simulink model "sf_msg_traffic_light"  (R2025b)
settings: Solver=FixedStepDiscrete  StartTime=0.0  StopTime=inf  FixedStep=.2  RelTol=1e-3  EnableMultiTasking=on
PostLoadFcn:
  | tl_gui('init', bdroot);
InitFcn:
  | tl_gui('reset', bdroot);
libraries: sf_msg_traffic_light_lib x6
CloseFcn:
  | tl_gui('close');
settings Model: PacingRate=0.500000  Creator=The MathWorks, Inc.  LastModifiedBy=The MathWorks, Inc.
settings SolverCC: AlgebraicLoopSolver=TrustRegion
settings DataIOCC: LimitDataPoints=on  SaveOutput=off  SignalLogging=off  DSMLogging=off  SaveTime=off  ReturnWorkspaceOutputs=off
settings OptimizationCC: ReuseModelBlockBuffer=off  LifeSpan=inf
settings DebuggingCC: UnconnectedInputMsg=warning  UnconnectedOutputMsg=warning  UnconnectedLineMsg=warning  AllowSymbolicDim=off  PregeneratedLibrarySubsystemCodeDiagnostic=none  SFUnexpectedBacktrackingDiag=warning  SFNoUnconditionalDefaultTransitionDiag=warning  SFExecutionAtInitializationDiag=none  ArithmeticOperatorsInVariantConditions=warning
settings HardwareCC: ProdBitPerPointer=32.0  ProdBitPerSizeT=32.0  ProdBitPerPtrDiffT=32.0  ProdLargestAtomicFloat=None  ProdIntDivRoundTo=Undefined  ProdEndianess=Unspecified  ProdWordSize=32.0  ProdHWDeviceType=32-bit Generic
settings ModelReferenceCC: EnableRefExpFcnMdlSchedulingChecks=on  PropagateSignalLabelsOutOfModel=off
settings SFSimCC: SimUseLocalCustomCode=off  CustomCodeUndefinedFunction=UseInterfaceOnly
settings RTWCC: GenCodeOnly=on  GenerateReport=on  RTWUseLocalCustomCode=off  LaunchReport=on  GPUComputeCapability=3.5
settings CodeAppCC: StateflowObjectComments=on
settings GRTTargetCC: TargetLangStandard=C89/C90 (ANSI)  UtilityFuncGeneration=Shared location
settings ConfigComp: CovMetricSettings=dw  CovSaveCumulativeToWorkspaceVar=on  CovSaveSingleToWorkspaceVar=on  CovExternalEMLEnable=off

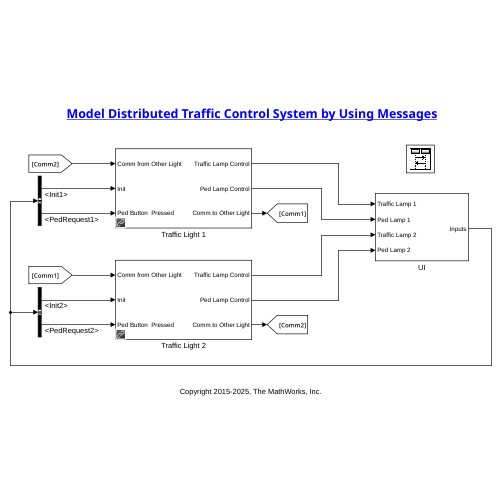
[thumbnail: Simulink's stored preview of the top-level diagram]
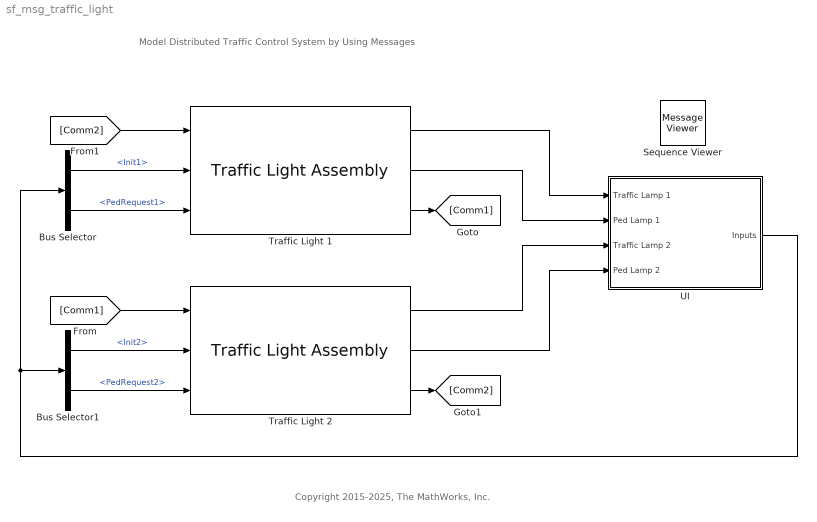
== system sf_msg_traffic_light ==
  note: Copyright 2015-2025, The MathWorks, Inc.
  note: Model Distributed Traffic Control System by Using Messages
  Bus Selector : BusSelector  OutputSignals=Init1,PedRequest1
  Bus Selector1 : BusSelector  OutputSignals=Init2,PedRequest2
  Sequence Viewer : MessageViewer  SavedRootId=#
  Traffic Light 1 : sf_msg_traffic_light_lib/Traffic Light Assembly  SystemSampleTime=-1  VariantActivationTime=update diagram  EmptyChoice=off  PassThrough=off  PassThroughVariantControl=(default)  EmptyChoiceVariantControl=(default)  AllowFlexibleInterface=on  Latency=0  AutoFrameSizeCalculation=off
  Traffic Light 2 : sf_msg_traffic_light_lib/Traffic Light Assembly  SystemSampleTime=-1  VariantActivationTime=update diagram  EmptyChoice=off  PassThrough=off  PassThroughVariantControl=(default)  EmptyChoiceVariantControl=(default)  AllowFlexibleInterface=on  Latency=0  AutoFrameSizeCalculation=off
  UI : Subsystem
  wires:
  Traffic Light 2/2 -> UI/4(Ped Lamp 2)
  Traffic Light 2/1 -> UI/3(Traffic Lamp 2)
  Traffic Light 1/2 -> UI/2(Ped Lamp 1)
  Traffic Light 1/1 -> UI/1(Traffic Lamp 1)
  Bus Selector/1 -> Traffic Light 1/2  "<Init1>"
  Bus Selector/2 -> Traffic Light 1/3  "<PedRequest1>"
  Bus Selector1/1 -> Traffic Light 2/2  "<Init2>"
  Bus Selector1/2 -> Traffic Light 2/3  "<PedRequest2>"
  UI/1(Inputs) -> Bus Selector1/1, Bus Selector/1
  Traffic Light 1/3 -> [Comm1]
  Traffic Light 2/3 -> [Comm2]
  [Comm2] -> Traffic Light 1/1
  [Comm1] -> Traffic Light 2/1

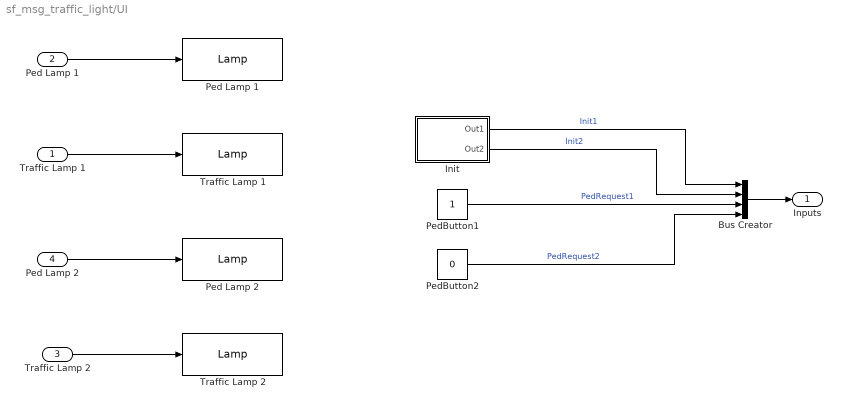
== system sf_msg_traffic_light/UI ==
  Traffic Lamp 1 : Inport
  Ped Lamp 1 : Inport  Port=2
  Traffic Lamp 2 : Inport  Port=3
  Ped Lamp 2 : Inport  Port=4
  " Ped Lamp 1" : sf_msg_traffic_light_lib/ Lamp  LampSelect=Ped Lamp 1
  " Ped Lamp 2" : sf_msg_traffic_light_lib/ Lamp  LampSelect=Ped Lamp 2
  " Traffic Lamp 1" : sf_msg_traffic_light_lib/ Lamp  LampSelect=Traffic Lamp 1
  " Traffic Lamp 2" : sf_msg_traffic_light_lib/ Lamp  LampSelect=Traffic Lamp 2
  Bus Creator : BusCreator  Inputs=4
  Init : Subsystem
  PedButton1 : Constant
  PedButton2 : Constant  Value=0
  Inputs : Outport  VectorParamsAs1DForOutWhenUnconnected=off
  wires:
  Init/1(Out1) -> Bus Creator/1  "Init1"
  Init/2(Out2) -> Bus Creator/2  "Init2"
  Bus Creator/1 -> Inputs/1
  Traffic Lamp 2/1 -> " Traffic Lamp 2"/1
  Ped Lamp 2/1 -> " Ped Lamp 2"/1
  Traffic Lamp 1/1 -> " Traffic Lamp 1"/1
  Ped Lamp 1/1 -> " Ped Lamp 1"/1
  PedButton1/1 -> Bus Creator/3  "PedRequest1"
  PedButton2/1 -> Bus Creator/4  "PedRequest2"

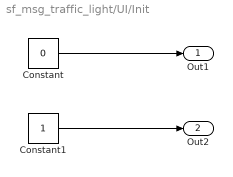
== system sf_msg_traffic_light/UI/Init ==
  Constant : Constant  Value=0
  Constant1 : Constant
  Out1 : Outport  VectorParamsAs1DForOutWhenUnconnected=off
  Out2 : Outport  Port=2  VectorParamsAs1DForOutWhenUnconnected=off
  wires:
  Constant/1 -> Out1/1
  Constant1/1 -> Out2/1
